simulink model "Highway_Assist"  (R2021a)
settings: Solver=VariableStepAuto  StartTime=0.0  StopTime=100  RelTol=1e-3
values from neighbouring files (symbols this model uses):
  Cf = 155494.663    [Highway_Assist_init.m]
  Cr = 1554494.663    [Highway_Assist_init.m]
  Iz = 1436.24    [Highway_Assist_init.m]
  lf = 1.165    [Highway_Assist_init.m]
  lr = 1.165    [Highway_Assist_init.m]
  m = 1140    [Highway_Assist_init.m]
  md = get_curvature(Vx, yaw_rate_pose, tRef)    [Highway_Assist_init.m]
  Ts = 0.1    [Highway_Assist_init.m]
  V_init = Vx    (= 25)    [Highway_Assist_init.m]
undefined symbols (not defined in the file or in its folder): sigbuilder_block
libraries: pid_lib x2, mpcadaslib x1
(part 2 of 2)

== system Highway_Assist/Sensor inputs/Radar sensor output/Signal Builder ==
  Demux : Demux  Tag=STV Demux  Outputs=2
      settings: DisplayOption=none
  FromWs : FromWorkspace  Tag=STV FromWs  VariableName=tuvar
      SigBuilderData=|
      | common.afterFinalStr = 'Extrapolate'
      | common.sampleTime = 0
      | dataSet.timeRange = [0 100]
      | dataSet.name = 'Group 1'
      | sbobj.Groups.Name = 'Group 1'
      | sbobj.Groups.Signals(1).Name = 'target'
      | sbobj.Groups.Signals(1).XData = [0 30 30 100]
      | sbobj.Groups.Signals(1).YData = [0 0 1 1]
      | sbobj.Groups.Signals(2).Name = 'no target'
      | sbobj.Groups.Signals(2).XData = [0 100]
      | sbobj.Groups.Signals(2).YData = [0 0]
      | sbobj.Groups.TimeRange = [0 100]
  target : Outport  Tag=STV Outport
  no target : Outport  Tag=STV Outport  Port=2
  wires:
  FromWs/1 -> Demux/1
  Demux/1 -> target/1
  Demux/2 -> no target/1

== system Highway_Assist/Controller/ACC Longitudinal control/Feedforward_Logic/If Action Subsystem ==
  Action Port : ActionPort  ActionPortLabel=if((u1 > 10))
  Constant : Constant
  Out1 : Outport
  wires:
  Constant/1 -> Out1/1

== system Highway_Assist/Controller/ACC Longitudinal control/Feedforward_Logic/If Action Subsystem1 ==
  Action Port : ActionPort  ActionPortLabel=elseif((u1 < 5))
  Constant : Constant  Value=3
  Out1 : Outport
  wires:
  Constant/1 -> Out1/1

== system Highway_Assist/Controller/ACC Longitudinal control/Feedforward_Logic/If Action Subsystem2 ==
  Action Port : ActionPort  ActionPortLabel=else
  Constant : Constant  Value=2
  Out1 : Outport
  wires:
  Constant/1 -> Out1/1

== matlab function Highway_Assist/Sensor inputs/Lateral control sensor inputs/Subsystem/MATLAB Function ==
  settings: updateMethod=DISCRETE  sampleTime=ts
  data: data parameter; seq output; steps parameter; t input; first output; next_t output
function [seq,first,next_t] = fcn(data,steps,t)
%#codegen
[seq,first,next_t] = mpcblock_preview('md',data,steps,t);

== stateflow chart Highway_Assist/Controller/ACC Longitudinal control/ACC State Logic/ACC State flow ==
  state Headway_control
    entry:en_man =false;
    en_vel = false;
    en_pos = true;
  state Velocity_control
    entry:en_man =false;
    en_vel = true;
    en_pos = false;
  state Manual_mode
    entry:en_man =true;
    en_vel = false;
    en_pos = false;
  Manual_mode -> Velocity_control [order 1] : [(ACC_enabled == 1) &&(Target_flag == 0)]
  Headway_control -> Velocity_control [order 2] : [(ACC_enabled == 1) & (Target_flag == 0) || V_host_mps > V_command_mps + 0.5 && after(30,sec)]
  Manual_mode -> Headway_control [order 2] : [(ACC_enabled == 1) && (Target_flag == 1)]
  (default) -> Manual_mode
  Velocity_control -> Manual_mode [order 1] : [(ACC_enabled == 0)]
  Headway_control -> Manual_mode [order 1] : [(ACC_enabled == 0)]
  Velocity_control -> Headway_control [order 2] : [(ACC_enabled == 1) & (Target_flag == 1) && after(30,sec)]
  data: ACC_enabled input; V_host_mps input; Target_flag input; en_man output; en_vel output; en_pos output; V_command_mps input

== stateflow chart Highway_Assist/HA mode manager/HA Mode manager/Chart ==
  state HA_off
    entry: en_manual = true;
    HA_active = false;
  state HA_ON
    state HA_ON
      entry: en_manual = false;
      HA_active = true;
      Hands_on = true;
    state HA_Off
      entry: en_manual = false;
      HA_active = true;
      Hands_on = false;
    (default) -> HA_ON.HA_ON
    HA_ON.HA_ON -> HA_Off : [(Hands_off_zone == 1)]
    HA_Off -> HA_ON.HA_ON : [(Hands_off_zone == 0)]
  (default) -> HA_off
  HA_ON -> HA_off : [(ACC_enable == 0)||(HA_available == 0)||(LCA_enable == 0)]
  HA_off -> HA_ON : [(ACC_enable == 1)&&(HA_available == 1)&&(LCA_enable == 1)]
  data: ACC_enable input; HA_available input; Hands_off_zone input; LCA_enable input; HA_active output; en_manual output; Hands_on output

== stateflow chart Highway_Assist/Controller/ACC Longitudinal control/Feedforward_Logic/Quadrant Chart ==
  state Quadrant2
    entry:
    quadrant = 2;
  state Quadrant1
    entry:
    quadrant = 1;
  state Quadrant3
    entry:
    quadrant = 3;
  state Quadrant4
    entry:
    quadrant = 4;
  (default) -> Quadrant1
  Quadrant1 -> (junction 6) : [((R < R_c) || (V_target_mps < V_host_mps)) && after(10,sec)]
  Quadrant2 -> (junction 6) : [((R > R_c) || (V_target_mps > V_host_mps)) && after(10,sec)]
  (junction 6) -> Quadrant2 [order 2] : [(R > R_c) && (V_target_mps < V_host_mps)]
  (junction 6) -> Quadrant1 [order 1] : [(R > R_c) && (V_target_mps > V_host_mps)]
  (junction 6) -> Quadrant3 [order 3] : [(R < R_c) && (V_target_mps < V_host_mps)]
  (junction 6) -> Quadrant4 [order 4] : [(R < R_c) && (V_target_mps > V_host_mps)]
  Quadrant3 -> (junction 6) : [((R > R_c) || (V_target_mps > V_host_mps)) && after(10,sec)]
  Quadrant4 -> (junction 6) : [((R > R_c) || (V_target_mps < V_host_mps)) && after(10,sec)]
  data: R_c input; R input; quadrant output; V_target_mps input; V_host_mps input
